simulink model "ibarra2321070902"  (R2026b)
settings: Solver=ode15s  StopTime=15  MaxStep=1E-2
libraries: slpidlib x2
settings Model: Creator=Chulis  LastModifiedBy=Ivana
settings DataIOCC: DSMLogging=off  ReturnWorkspaceOutputs=off  SaveOutput=off  SignalLogging=off  TimeSaveName=t
settings DebuggingCC: AlgebraicLoopMsg=none  ArtificialAlgebraicLoopMsg=none  MaxConsecutiveZCsMsg=none  OperatingPointInterfaceChecksumMismatchMsg=none

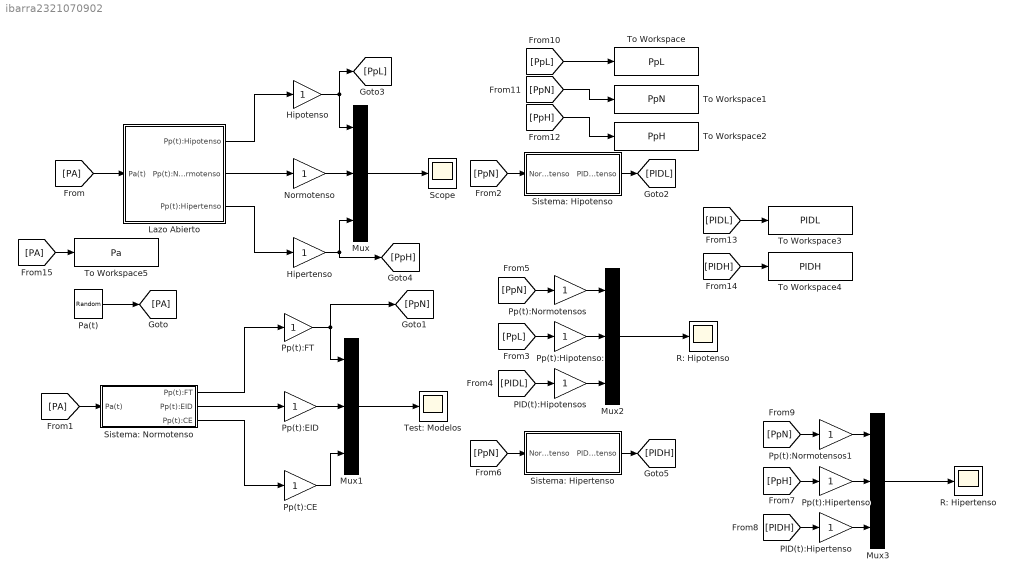
== system ibarra2321070902 ==
  Hipertenso : Gain
  Hipotenso : Gain
  Lazo Abierto : Subsystem
  Mux{,1..3} (4 alike) : Mux  Inputs=3
  Normotenso : Gain
  PID(t):Hipertenso : Gain
  PID(t):Hipotensos : Gain
  Pa(t) : UniformRandomNumber  Minimum=-0.2  Seed=106  SampleTime=0.1
  Pp(t):CE : Gain
  Pp(t):EID : Gain
  Pp(t):FT : Gain
  Pp(t):Hipertenso : Gain
  Pp(t):Hipotenso: : Gain
  Pp(t):Normotensos : Gain
  Pp(t):Normotensos1 : Gain
  R: Hipertenso : Scope
      settings: ActiveDisplayYMinimum=-0.489551907510661  ActiveDisplayYMaximum=1.2815596794800641  DataLoggingVariableName=ScopeData3
  R: Hipotenso : Scope
      settings: ActiveDisplayYMinimum=-0.55245363787357216  ActiveDisplayYMaximum=1.3294930978190262  DataLoggingVariableName=ScopeData2
  Scope : Scope
      settings: ActiveDisplayYMinimum=-0.55245363787357216  ActiveDisplayYMaximum=1.3294930978190262
  Sistema: Hipertenso : Subsystem
  Sistema: Hipotenso : Subsystem
  Sistema: Normotenso : Subsystem
  Test: Modelos : Scope
      settings: ActiveDisplayYMinimum=-0.43154608386478566  ActiveDisplayYMaximum=1.2111656073854709
  To Workspace : ToWorkspace  VariableName=PpL  SampleTime=-1
  To Workspace1 : ToWorkspace  VariableName=PpN  SampleTime=-1
  To Workspace2 : ToWorkspace  VariableName=PpH  SampleTime=-1
  To Workspace3 : ToWorkspace  VariableName=PIDL  SampleTime=-1
  To Workspace4 : ToWorkspace  VariableName=PIDH  SampleTime=-1
  To Workspace5 : ToWorkspace  VariableName=Pa  SampleTime=-1
  wires:
  Pa(t)/1 -> [PA]
  [PA] -> Lazo Abierto/1(Pa(t))
  Lazo Abierto/1(Pp(t):Hipotenso) -> Hipotenso/1
  Hipotenso/1 -> [PpL], Mux/1
  Lazo Abierto/2(Pp(t):Normotenso) -> Normotenso/1
  Normotenso/1 -> Mux/2
  Lazo Abierto/3(Pp(t):Hipertenso) -> Hipertenso/1
  Hipertenso/1 -> [PpH], Mux/3
  Mux/1 -> Scope/1
  [PA] -> Sistema: Normotenso/1(Pa(t))
  Sistema: Normotenso/2(Pp(t):EID) -> Pp(t):EID/1
  Pp(t):CE/1 -> Mux1/3
  Sistema: Normotenso/1(Pp(t):FT) -> Pp(t):FT/1
  Pp(t):FT/1 -> [PpN], Mux1/1
  Pp(t):EID/1 -> Mux1/2
  Sistema: Normotenso/3(Pp(t):CE) -> Pp(t):CE/1
  Mux1/1 -> Test: Modelos/1
  [PpN] -> Sistema: Hipotenso/1(Normotenso)
  Sistema: Hipotenso/1(PID(t):Hipotenso) -> [PIDL]
  [PpN] -> Pp(t):Normotensos/1
  [PpL] -> Pp(t):Hipotenso:/1
  [PIDL] -> PID(t):Hipotensos/1
  Mux2/1 -> R: Hipotenso/1
  Pp(t):Hipotenso:/1 -> Mux2/2
  PID(t):Hipotensos/1 -> Mux2/3
  Pp(t):Normotensos/1 -> Mux2/1
  [PpN] -> Sistema: Hipertenso/1(Normotenso)
  Sistema: Hipertenso/1(PID(t):Hipertenso) -> [PIDH]
  PID(t):Hipertenso/1 -> Mux3/3
  [PIDH] -> PID(t):Hipertenso/1
  [PpH] -> Pp(t):Hipertenso/1
  [PpN] -> Pp(t):Normotensos1/1
  Pp(t):Normotensos1/1 -> Mux3/1
  Pp(t):Hipertenso/1 -> Mux3/2
  Mux3/1 -> R: Hipertenso/1
  [PpL] -> To Workspace/1
  [PpN] -> To Workspace1/1
  [PpH] -> To Workspace2/1
  [PIDL] -> To Workspace3/1
  [PIDH] -> To Workspace4/1
  [PA] -> To Workspace5/1

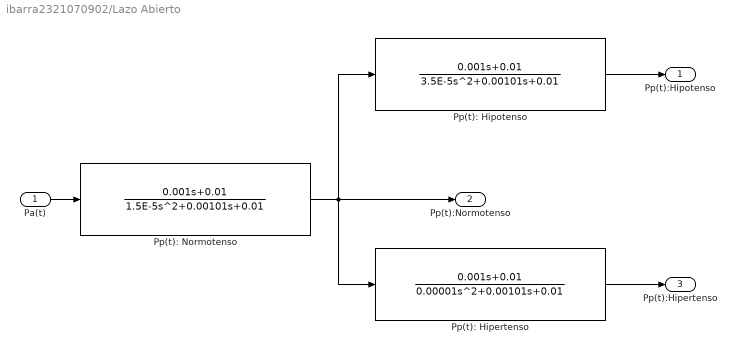
== system ibarra2321070902/Lazo Abierto ==
  Pa(t) : Inport
  Pp(t): Hipertenso : TransferFcn  Numerator=[0.001,0.01]  Denominator=[0.00001,0.00101,0.01]
  Pp(t): Hipotenso : TransferFcn  Numerator=[0.001,0.01]  Denominator=[3.5E-5,0.00101,0.01]
  Pp(t): Normotenso : TransferFcn  Numerator=[0.001,0.01]  Denominator=[1.5E-5,0.00101,0.01]
  Pp(t):Hipotenso : Outport
  Pp(t):Normotenso : Outport  Port=2
  Pp(t):Hipertenso : Outport  Port=3
  wires:
  Pa(t)/1 -> Pp(t): Normotenso/1
  Pp(t): Normotenso/1 -> Pp(t):Normotenso/1, Pp(t): Hipertenso/1, Pp(t): Hipotenso/1
  Pp(t): Hipotenso/1 -> Pp(t):Hipotenso/1
  Pp(t): Hipertenso/1 -> Pp(t):Hipertenso/1

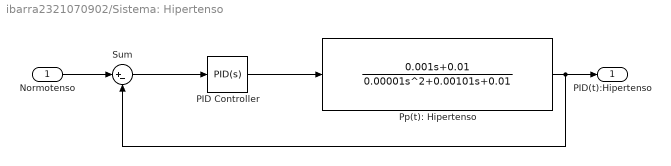
== system ibarra2321070902/Sistema: Hipertenso ==
  Normotenso : Inport
  PID Controller : slpidlib/PID Controller  Controller=PID  Form=Parallel  TimeDomain=Continuous-time  UseExternalTs=off  SampleTime=-1  IntegratorMethod=Forward Euler  FilterMethod=Forward Euler  ControllerParametersSource=internal  P=129.9786  I=312762.8587  UseKiTs=off  D=0.0017461  UseExternalDerivativeSource=off  N=49610.1327  UseFilter=on  TunerSelectOption=Transfer Function Based (PID Tuner App)  InitialConditionSource=internal  InitialConditionForIntegrator=0  InitialConditionForFilter=0  DifferentiatorICPrevScaledInput=0  ExternalReset=none  TrackingMode=off  Kt=1  LimitOutput=off  SatLimitsSource=internal  UpperSaturationLimit=inf  LowerSaturationLimit=-inf  LinearizeAsGain=on  AntiWindupMode=none  Kb=1  LimitIntegrator=off  UpperIntegratorSaturationLimit=inf  LowerIntegratorSaturationLimit=-inf  POutMin=[]  POutMax=[]  IOutMin=[]  IOutMax=[]  DOutMin=[]  DOutMax=[]  NOutMin=[]  NOutMax=[]  SumOutMin=[]  SumOutMax=[]  SaturationOutMin=[]  SaturationOutMax=[]  PParamMin=[]  PParamMax=[]  IParamMin=[]  IParamMax=[]  DParamMin=[]  DParamMax=[]  NParamMin=[]  NParamMax=[]  KbParamMin=[]  KbParamMax=[]  KtParamMin=[]  KtParamMax=[]  KbOutMin=[]  KbOutMax=[]  KtOutMin=[]  KtOutMax=[]  IntegratorOutMin=[]  IntegratorOutMax=[]  FilterOutMin=[]  FilterOutMax=[]  SumI1OutMin=[]  SumI1OutMax=[]  SumI2OutMin=[]  SumI2OutMax=[]  SumI3OutMin=[]  SumI3OutMax=[]  SumI4OutMin=[]  SumI4OutMax=[]  SumDOutMin=[]  SumDOutMax=[]  DifferentiatorOutMin=[]  DifferentiatorOutMax=[]  FilterDiffOutCoefMin=[]  FilterDiffOutCoefMax=[]  ReciprocalOutMin=[]  ReciprocalOutMax=[]  SumDenOutMin=[]  SumDenOutMax=[]  SumNumOutMin=[]  SumNumOutMax=[]  DivideOutMin=[]  DivideOutMax=[]  UdiffTsProdOutMin=[]  UdiffTsProdOutMax=[]  NTsProdOutMin=[]  NTsProdOutMax=[]  UintegralTsProdOutMin=[]  UintegralTsProdOutMax=[]  UngainTsProdOutMin=[]  UngainTsProdOutMax=[]  ClampingZeroOutDataTypeStr=Inherit: Inherit via back propagation  ClampingZeroOutMin=[]  ClampingZeroOutMax=[]  FilterDenConstantOutDataTypeStr=Inherit: Inherit via back propagation  FilterDenConstantOutMin=[]  FilterDenConstantOutMax=[]  PCopyOutDataTypeStr=Inherit: Inherit via back propagation  PCopyOutMin=[]  PCopyOutMax=[]  NCopyOutDataTypeStr=Inherit: Inherit via back propagation  NCopyOutMin=[]  NCopyOutMax=[]  IntegratorContinuousStateAttributes=''  IntegratorStateMustResolveToSignalObject=off  IntegratorRTWStateStorageClass=Auto  FilterContinuousStateAttributes=''  FilterStateMustResolveToSignalObject=off  FilterRTWStateStorageClass=Auto  ParallelPVariant=InternalParameters  IdealPVariant=Disabled  IVariant=InternalParameters  DVariant=InternalParameters  IntegratorVariant=Continuous  SatVariant=Disabled  AWVariant=Passthrough  PCopyVariant=Disabled  TRVariant=Disabled  FdbkBlocksVariant=Forward  IdealPFdbkVariant=Disabled  SatFdbkVariant=Disabled  DerivativeFilterVariant=ContFilter  NVariant=InternalParameters  NCopyVariant=Disabled  FilterICVariant=InternalICsFilter  IntegratorICVariant=InternalICs  ExternalResetVariant=Disabled  TRSumVariant=Passthrough  SumFdbkVariant=Disabled  SumVariant=Sum_PID  TsampFilterVariant=InternalTs  TsampNgainVariant=Passthrough  TsampIntegralVariant=Disabled_SignalSpec  ExternalSaturationOutDataTypeStr=Inherit: Same as second input  DerivativeSourceVariant=ErrorSignal  PreIntVariant=InternalPreInt
  Pp(t): Hipertenso : TransferFcn  Numerator=[0.001,0.01]  Denominator=[0.00001,0.00101,0.01]
  Sum : Sum  Inputs=|+-
  PID(t):Hipertenso : Outport
  wires:
  Normotenso/1 -> Sum/1
  Sum/1 -> PID Controller/1
  PID Controller/1 -> Pp(t): Hipertenso/1
  Pp(t): Hipertenso/1 -> PID(t):Hipertenso/1, Sum/2

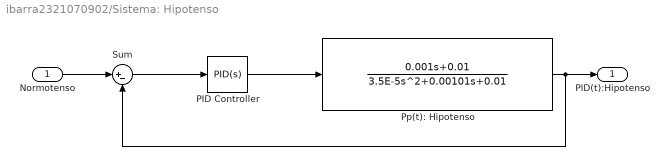
== system ibarra2321070902/Sistema: Hipotenso ==
  Normotenso : Inport
  PID Controller : slpidlib/PID Controller  Controller=PID  Form=Parallel  TimeDomain=Continuous-time  UseExternalTs=off  SampleTime=-1  IntegratorMethod=Forward Euler  FilterMethod=Forward Euler  ControllerParametersSource=internal  P=458.4826  I=1112094.7355  UseKiTs=off  D=0.0062671  UseExternalDerivativeSource=off  N=50057.6251  UseFilter=on  TunerSelectOption=Transfer Function Based (PID Tuner App)  InitialConditionSource=internal  InitialConditionForIntegrator=0  InitialConditionForFilter=0  DifferentiatorICPrevScaledInput=0  ExternalReset=none  TrackingMode=off  Kt=1  LimitOutput=off  SatLimitsSource=internal  UpperSaturationLimit=inf  LowerSaturationLimit=-inf  LinearizeAsGain=on  AntiWindupMode=none  Kb=1  LimitIntegrator=off  UpperIntegratorSaturationLimit=inf  LowerIntegratorSaturationLimit=-inf  POutMin=[]  POutMax=[]  IOutMin=[]  IOutMax=[]  DOutMin=[]  DOutMax=[]  NOutMin=[]  NOutMax=[]  SumOutMin=[]  SumOutMax=[]  SaturationOutMin=[]  SaturationOutMax=[]  PParamMin=[]  PParamMax=[]  IParamMin=[]  IParamMax=[]  DParamMin=[]  DParamMax=[]  NParamMin=[]  NParamMax=[]  KbParamMin=[]  KbParamMax=[]  KtParamMin=[]  KtParamMax=[]  KbOutMin=[]  KbOutMax=[]  KtOutMin=[]  KtOutMax=[]  IntegratorOutMin=[]  IntegratorOutMax=[]  FilterOutMin=[]  FilterOutMax=[]  SumI1OutMin=[]  SumI1OutMax=[]  SumI2OutMin=[]  SumI2OutMax=[]  SumI3OutMin=[]  SumI3OutMax=[]  SumI4OutMin=[]  SumI4OutMax=[]  SumDOutMin=[]  SumDOutMax=[]  DifferentiatorOutMin=[]  DifferentiatorOutMax=[]  FilterDiffOutCoefMin=[]  FilterDiffOutCoefMax=[]  ReciprocalOutMin=[]  ReciprocalOutMax=[]  SumDenOutMin=[]  SumDenOutMax=[]  SumNumOutMin=[]  SumNumOutMax=[]  DivideOutMin=[]  DivideOutMax=[]  UdiffTsProdOutMin=[]  UdiffTsProdOutMax=[]  NTsProdOutMin=[]  NTsProdOutMax=[]  UintegralTsProdOutMin=[]  UintegralTsProdOutMax=[]  UngainTsProdOutMin=[]  UngainTsProdOutMax=[]  ClampingZeroOutDataTypeStr=Inherit: Inherit via back propagation  ClampingZeroOutMin=[]  ClampingZeroOutMax=[]  FilterDenConstantOutDataTypeStr=Inherit: Inherit via back propagation  FilterDenConstantOutMin=[]  FilterDenConstantOutMax=[]  PCopyOutDataTypeStr=Inherit: Inherit via back propagation  PCopyOutMin=[]  PCopyOutMax=[]  NCopyOutDataTypeStr=Inherit: Inherit via back propagation  NCopyOutMin=[]  NCopyOutMax=[]  IntegratorContinuousStateAttributes=''  IntegratorStateMustResolveToSignalObject=off  IntegratorRTWStateStorageClass=Auto  FilterContinuousStateAttributes=''  FilterStateMustResolveToSignalObject=off  FilterRTWStateStorageClass=Auto  ParallelPVariant=InternalParameters  IdealPVariant=Disabled  IVariant=InternalParameters  DVariant=InternalParameters  IntegratorVariant=Continuous  SatVariant=Disabled  AWVariant=Passthrough  PCopyVariant=Disabled  TRVariant=Disabled  FdbkBlocksVariant=Forward  IdealPFdbkVariant=Disabled  SatFdbkVariant=Disabled  DerivativeFilterVariant=ContFilter  NVariant=InternalParameters  NCopyVariant=Disabled  FilterICVariant=InternalICsFilter  IntegratorICVariant=InternalICs  ExternalResetVariant=Disabled  TRSumVariant=Passthrough  SumFdbkVariant=Disabled  SumVariant=Sum_PID  TsampFilterVariant=InternalTs  TsampNgainVariant=Passthrough  TsampIntegralVariant=Disabled_SignalSpec  ExternalSaturationOutDataTypeStr=Inherit: Same as second input  DerivativeSourceVariant=ErrorSignal  PreIntVariant=InternalPreInt
  Pp(t): Hipotenso : TransferFcn  Numerator=[0.001,0.01]  Denominator=[3.5E-5,0.00101,0.01]
  Sum : Sum  Inputs=|+-
  PID(t):Hipotenso : Outport
  wires:
  Normotenso/1 -> Sum/1
  Sum/1 -> PID Controller/1
  PID Controller/1 -> Pp(t): Hipotenso/1
  Pp(t): Hipotenso/1 -> PID(t):Hipotenso/1, Sum/2

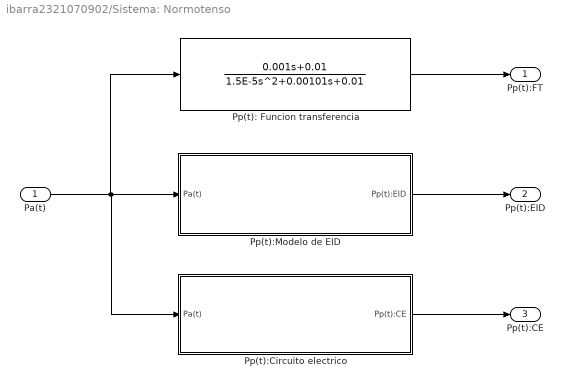
== system ibarra2321070902/Sistema: Normotenso ==
  Pa(t) : Inport
  "Pp(t): Funcion transferencia " : TransferFcn  Numerator=[0.001,0.01]  Denominator=[1.5E-5,0.00101,0.01]
  Pp(t):Circuito electrico : Subsystem
  Pp(t):Modelo de EID : Subsystem
  Pp(t):FT : Outport
  Pp(t):EID : Outport  Port=2
  Pp(t):CE : Outport  Port=3
  wires:
  Pa(t)/1 -> Pp(t):Circuito electrico/1(Pa(t)), Pp(t):Modelo de EID/1(Pa(t)), "Pp(t): Funcion transferencia "/1
  "Pp(t): Funcion transferencia "/1 -> Pp(t):FT/1
  Pp(t):Modelo de EID/1(Pp(t):EID) -> Pp(t):EID/1
  Pp(t):Circuito electrico/1(Pp(t):CE) -> Pp(t):CE/1

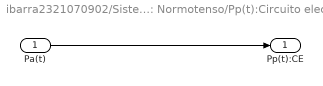
== system ibarra2321070902/Sistema: Normotenso/Pp(t):Circuito electrico ==
  Pa(t) : Inport
  Pp(t):CE : Outport
  wires:
  Pa(t)/1 -> Pp(t):CE/1

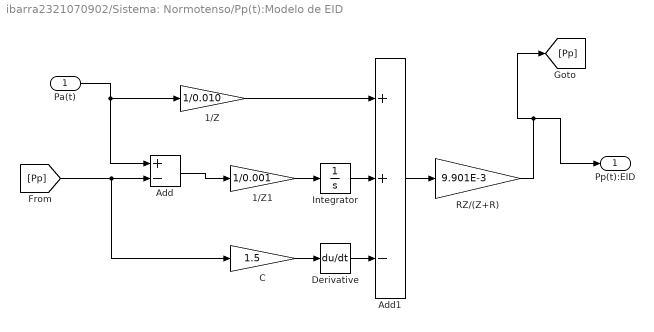
== system ibarra2321070902/Sistema: Normotenso/Pp(t):Modelo de EID ==
  Pa(t) : Inport
  1/Z : Gain  Gain=1/0.010
  1/Z1 : Gain  Gain=1/0.001
  Add : Sum  Inputs=+-
  Add1 : Sum  Inputs=++-
  C : Gain  Gain=1.5
  Derivative : Derivative
  Integrator : Integrator
  RZ/(Z+R) : Gain  Gain=9.901E-3
  Pp(t):EID : Outport
  wires:
  Pa(t)/1 -> Add/1, 1/Z/1
  RZ/(Z+R)/1 -> [Pp], Pp(t):EID/1
  [Pp] -> C/1, Add/2
  Add/1 -> 1/Z1/1
  Add1/1 -> RZ/(Z+R)/1
  1/Z/1 -> Add1/1
  1/Z1/1 -> Integrator/1
  Integrator/1 -> Add1/2
  C/1 -> Derivative/1
  Derivative/1 -> Add1/3
